simulink model "Y3Tiltrotor_sim3_INDI"  (R2025a)
settings: Solver=ode4  StartTime=0.0  StopTime=70  FixedStep=uavParam.sampleTime  RelTol=1e-3
PreLoadFcn:
  | filepath  = fileparts(get_param(bdroot, 'FileName'))
  | cd(filepath);
InitFcn:
  | Init_sim_INDI;
values from neighbouring files (symbols this model uses):
  control = struct    [Init_sim_INDI.m]
  env = struct    [InitData.m]
  flightState = struct    [Init_sim_INDI.m]
  FWSpeed0 = 15    [Init_sim_INDI.m]
  k_lpf_p = 50    [Init_sim_INDI.m]
  k_lpf_q = 80    [Init_sim_INDI.m]
  k_lpf_r = 5    [Init_sim_INDI.m]
  k_lpf_u = 10    [Init_sim_INDI.m]
  k_lpf_v = 1    [Init_sim_INDI.m]
  k_lpf_w = 50    [Init_sim_INDI.m]
  k_p = 5    [Init_sim_INDI.m]
  k_q = 20    [Init_sim_INDI.m]
  k_r = 1.5    [Init_sim_INDI.m]
  k_u = 0.5    [Init_sim_INDI.m]
  k_v = 0.5    [Init_sim_INDI.m]
  k_w = 2    [Init_sim_INDI.m]
  uavParam = struct    [InitData.m]
undefined symbols (not defined in the file or in its folder): ControlSampleTime, F, Light, MIL, Newton, Raphson
libraries: slpidlib x28, SignalEditorBlockLib x12, simulink x6, aerolibtransform2 x3, sharedtransform x3, robotcorelib x3, matrix_library x3, aerolibasang x2, aerolibutil x2, aerolibwind2 x2, shared6dof x1, aerolibatmos2 x1
(part 7 of 7)

== matlab function Y3Tiltrotor_sim3_INDI/Y3 Tiltrotor Aircraft Model/Subsystem/Aerodynamic Forces and Moments/Compute Body Frame Aerodynamic Forces and Moments/Wind frame F& M/Longitudinal Channel/CD/CD(delta_e) ==
  data: delta_e input; CD_delta_e output
function CD_delta_e = fcn_CD_delta_e(delta_e)

    c1 = 0.000707;
    c2 = 0.000057;
    c3 = 0.013601;
    c4 = 0.101850;
    c5 = 1.443831;
    c6 = 56.012704;
    c7 = 0.000024;
    c8 = 0.101300;
    c9 = -0.021731;
    c10 = -3.024408;
    c11 = 61.266062;

    CD_delta_e = zeros(size(delta_e));

    idx_pos = delta_e >= 0;
    if any(idx_pos)
        delta_e_pos = delta_e(idx_pos);
        CD_delta_e(idx_pos) = (1+tanh(c1*(47.4^2-delta_e_pos.^2)))/(1+tanh(c1*47.4^2)).*(c2*delta_e_pos.^2)...
            +(1-(1+tanh(c1*(47.4^2-delta_e_pos.^2)))/(1+tanh(c1*47.4^2))).*(c3+c4*sin(c5*pi/180*delta_e_pos+c6).^2);
    end

    idx_neg = delta_e < 0;
    if any(idx_neg)
        delta_e_neg = delta_e(idx_neg);
        CD_delta_e(idx_neg) = (1+tanh(c1*(47.4^2-delta_e_neg.^2)))/(1+tanh(c1*47.4^2)).*(c7*delta_e_neg.^2)...
            +(1-(1+tanh(c1*(47.4^2-delta_e_neg.^2)))/(1+tanh(c1*47.4^2))).*(c8+c9*sin(c10*pi/180*delta_e_neg+c11).^2);
    end
    
end
